simulink model "ElectricVehicleThermalManagementWithHeatPump"  (R2024b)
settings: Solver=VariableStepAuto  StartTime=0.0  StopTime=3600  RelTol=1e-3  AbsTol=1e-3
PreLoadFcn:
  | init_nmpc
InitFcn:
  | init_nmpc
model workspace: external: MATLAB File ElectricVehicleThermalManagementWithHeatPumpParameters.m (data not in the file)
values from neighbouring files (symbols this model uses):
  battery_C1_LUT = [1913.6 12447 30609 ... (first row only)    [ElectricVehicleThermalManagementWithHeatPumpParameters.m]
  battery_capacity_LUT = [280.081 276.25 276.392]    [ElectricVehicleThermalManagementWithHeatPumpParameters.m]
  battery_cell_cp = 795    [ElectricVehicleThermalManagementWithHeatPumpParameters.m]
  battery_cell_mass = 2.5    [ElectricVehicleThermalManagementWithHeatPumpParameters.m]
  battery_Em_LUT = [3.4966 3.5057 3.5148 ... (first row only)    [ElectricVehicleThermalManagementWithHeatPumpParameters.m]
  battery_N_cells = 20    [ElectricVehicleThermalManagementWithHeatPumpParameters.m]
  battery_Qe_init = 0    [ElectricVehicleThermalManagementWithHeatPumpParameters.m]
  battery_R0_LUT = [0.0117 0.0085 0.009 ... (first row only)    [ElectricVehicleThermalManagementWithHeatPumpParameters.m]
  battery_R1_LUT = [0.0109 0.0029 0.0013 ... (first row only)    [ElectricVehicleThermalManagementWithHeatPumpParameters.m]
  battery_SOC_LUT = [0; 0.1; 0.25; 0.5; 0.75; 0.9; 1]    [ElectricVehicleThermalManagementWithHeatPumpParameters.m]
  battery_T_init = -10    [ElectricVehicleThermalManagementWithHeatPumpParameters.m]
  battery_temperature_LUT = [5 20 40]    [ElectricVehicleThermalManagementWithHeatPumpParameters.m]
  cabin_duct_area = 0.04    [ElectricVehicleThermalManagementWithHeatPumpParameters.m]
  cabin_T_init = -10    [ElectricVehicleThermalManagementWithHeatPumpParameters.m]
  chiller_area_primary = 0.43982297150257105    (= 0.439822971503)    [ElectricVehicleThermalManagementWithHeatPumpParameters.m]
  chiller_N_baffles = 3    [ElectricVehicleThermalManagementWithHeatPumpParameters.m]
  chiller_N_tubes = 100    [ElectricVehicleThermalManagementWithHeatPumpParameters.m]
  chiller_tube_D = 0.0035    [ElectricVehicleThermalManagementWithHeatPumpParameters.m]
  chiller_tube_L = 0.4    [ElectricVehicleThermalManagementWithHeatPumpParameters.m]
  chiller_wall_conductivity = 240    [ElectricVehicleThermalManagementWithHeatPumpParameters.m]
  chiller_wall_thickness = 0.0001    [ElectricVehicleThermalManagementWithHeatPumpParameters.m]
  cond_evap_air_area_flow = 0.3906    [ElectricVehicleThermalManagementWithHeatPumpParameters.m]
  cond_evap_air_area_primary = 1.4834999999999998    (= 1.4835)    [ElectricVehicleThermalManagementWithHeatPumpParameters.m]
  cond_evap_W = 0.015    [ElectricVehicleThermalManagementWithHeatPumpParameters.m]
  cond_evap_wall_conductivity = 240    [ElectricVehicleThermalManagementWithHeatPumpParameters.m]
  cond_evap_wall_thickness = 0.0001    [ElectricVehicleThermalManagementWithHeatPumpParameters.m]
  coolant_channel_D = 0.0092    [ElectricVehicleThermalManagementWithHeatPumpParameters.m]
  coolant_pipe_D = 0.019    [ElectricVehicleThermalManagementWithHeatPumpParameters.m]
  coolant_T_init = -10    [ElectricVehicleThermalManagementWithHeatPumpParameters.m]
  coolant_tank_area = 0.0121    [ElectricVehicleThermalManagementWithHeatPumpParameters.m]
  coolant_tank_volume = 1.25    [ElectricVehicleThermalManagementWithHeatPumpParameters.m]
  coolant_valve_D_ratio_max = 0.95    [ElectricVehicleThermalManagementWithHeatPumpParameters.m]
  coolant_valve_D_ratio_min = 0.001    [ElectricVehicleThermalManagementWithHeatPumpParameters.m]
  coolant_valve_displacement = 0.0063    [ElectricVehicleThermalManagementWithHeatPumpParameters.m]
  coolant_valve_S_max = 0.0053    [ElectricVehicleThermalManagementWithHeatPumpParameters.m]
  evaporator_air_area_flow = 0.12    [ElectricVehicleThermalManagementWithHeatPumpParameters.m]
  evaporator_air_area_primary = 0.4323    [ElectricVehicleThermalManagementWithHeatPumpParameters.m]
  evaporator_W = 0.015    [ElectricVehicleThermalManagementWithHeatPumpParameters.m]
  evaporator_wall_conductivity = 240    [ElectricVehicleThermalManagementWithHeatPumpParameters.m]
  evaporator_wall_thickness = 0.0001    [ElectricVehicleThermalManagementWithHeatPumpParameters.m]
  expansion_valve_D_ratio_max = 0.9    [ElectricVehicleThermalManagementWithHeatPumpParameters.m]
  hex_area_primary = 0.070371675440411369    (= 0.0703716754404)    [ElectricVehicleThermalManagementWithHeatPumpParameters.m]
  hex_N_tubes = 64    [ElectricVehicleThermalManagementWithHeatPumpParameters.m]
  hex_tube_D = 0.0035    [ElectricVehicleThermalManagementWithHeatPumpParameters.m]
  hex_wall_conductivity = 240    [ElectricVehicleThermalManagementWithHeatPumpParameters.m]
  hex_wall_thickness = 0.0001    [ElectricVehicleThermalManagementWithHeatPumpParameters.m]
  inner_cond_air_area_flow = 0.1953    [ElectricVehicleThermalManagementWithHeatPumpParameters.m]
  inner_cond_air_area_primary = 0.99520000000000008    (= 0.9952)    [ElectricVehicleThermalManagementWithHeatPumpParameters.m]
  inner_cond_W = 0.02    [ElectricVehicleThermalManagementWithHeatPumpParameters.m]
  inner_cond_wall_conductivity = 240    [ElectricVehicleThermalManagementWithHeatPumpParameters.m]
  inner_cond_wall_thickness = 0.0001    [ElectricVehicleThermalManagementWithHeatPumpParameters.m]
  pump_speed_max = 1000    [ElectricVehicleThermalManagementWithHeatPumpParameters.m]
  radiator_air_area_flow = 0.097499999999999989    (= 0.0975)    [ElectricVehicleThermalManagementWithHeatPumpParameters.m]
  radiator_air_area_primary = 0.43687499999999996    (= 0.436875)    [ElectricVehicleThermalManagementWithHeatPumpParameters.m]
  radiator_W = 0.015    [ElectricVehicleThermalManagementWithHeatPumpParameters.m]
  radiator_wall_conductivity = 240    [ElectricVehicleThermalManagementWithHeatPumpParameters.m]
  radiator_wall_thickness = 0.0001    [ElectricVehicleThermalManagementWithHeatPumpParameters.m]
  refrigerant_p_init = 0.2    [ElectricVehicleThermalManagementWithHeatPumpParameters.m]
  refrigerant_pipe_D = 0.01    [ElectricVehicleThermalManagementWithHeatPumpParameters.m]
  refrigerant_valve_D_ratio_max = 0.95    [ElectricVehicleThermalManagementWithHeatPumpParameters.m]
  refrigerant_valve_displacement = 0.005    [ElectricVehicleThermalManagementWithHeatPumpParameters.m]
libraries: fl_lib x227, nesl_utility x162, SimscapeFluids_lib x30, LiBatteryElements_lib x16, slpidlib x3, SignalEditorBlockLib x1
(part 4 of 13)

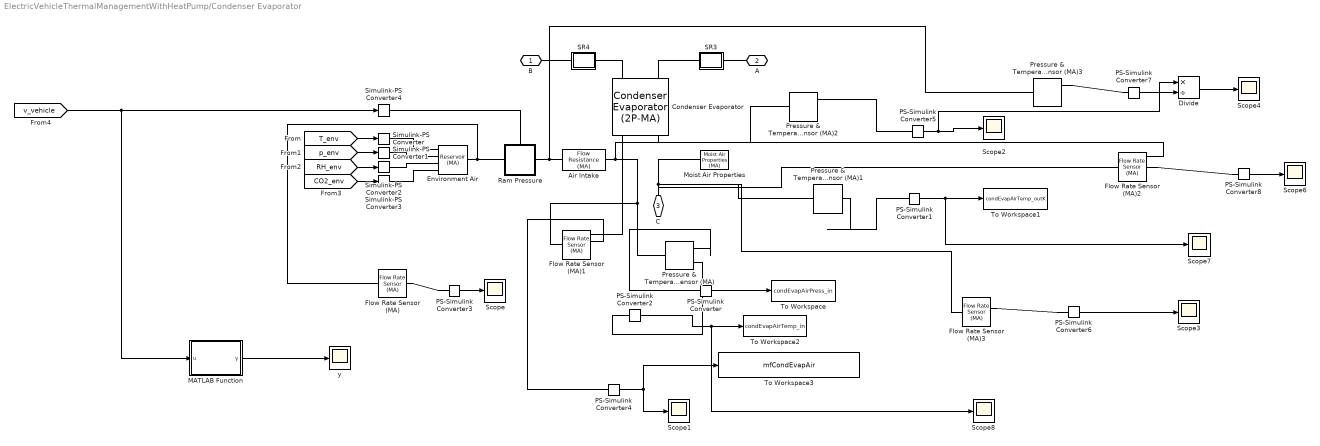
== system ElectricVehicleThermalManagementWithHeatPump/Condenser Evaporator ==
  Air Intake : fl_lib/Moist Air/Elements/Flow Resistance (MA)  delta_p_nominal=5e-4 MPa  mdot_nominal=1 kg/s  rho_nominal=1.2 kg/m^3  area=cabin_duct_area m^2  laminar_fraction=1e-3
  Condenser Evaporator : SimscapeFluids_lib/Heat Exchangers/Two-Phase Fluid - Moist Air/Condenser Evaporator (2P-MA)  flow_arrangement=fluids.heat_exchangers.enum.FlowArrangement2PMA.Cross  cross_flow_arrangement=fluids.heat_exchangers.enum.CrossFlowArrangement2PMA.UnmixedUnmixed  R_wall=cond_evap_wall_thickness / cond_evap_air_area_primary / cond_evap_wall_conductivity K/W  area_A1=pi * refrigerant_pipe_D^2 / 4 m^2  area_B1=pi * refrigerant_pipe_D^2 / 4 m^2  area_A2=cabin_duct_area m^2  area_B2=cabin_duct_area m^2  tube_num_2P=cond_evap_N_tubes  tube_length_2P=cond_evap_L m  tube_cross_section_2P=fluids.heat_exchangers.enum.TubeCrossSection.Rectangular  tube_diameter_2P=0.1 m  tube_width_2P=cond_evap_W m  tube_height_2P=cond_evap_tube_H m  tube_inner_diameter_2P=0.05 m  tube_outer_diameter_2P=0.1 m  tube_flow_area_2P=0.01 m^2  tube_wetted_perimeter_2P=0.4 m  tube_heat_perimeter_2P=0.4 m  tube_pressure_loss_spec_2P=fluids.heat_exchangers.enum.TubePressureLossSpec2P.Haaland  tube_loss_coeff_2P=10  tube_local_pressure_loss_spec_2P=fluids.heat_exchangers.enum.LocalLossSpec.AggregateLength  tube_length_add_2P=cond_evap_tube_Leq m  tube_local_loss_coefficient_2P=0.1  tube_roughness_pressure_2P=15e-6 m  tube_Re_lam_pressure_2P=2000  tube_Re_tur_pressure_2P=4000  tube_shape_factor_generic_2P=64  tube_heat_coeff_spec_2P=fluids.heat_exchangers.enum.TubeHeatCoeffSpec2P.GneilinskiCavalliniZecchin  tube_colburn_coeff_liq_2P=[.023, .8, .33]  tube_colburn_coeff_mix_2P=[.05, .8, .33]  tube_colburn_coeff_vap_2P=[.023, .8, .33]  tube_roughness_heat_2P=15e-6 m  tube_Re_lam_heat_2P=2000  tube_Re_tur_heat_2P=4000  tube_Nu_lam_generic_2P=3.66  fouling_factor_2P=0.1 m^2*K/kW  fin_area_2P=cond_evap_tube_area_webs m^2  fin_efficiency_2P=0.6  energy_spec_2P=foundation.enum.energy_spec.void_fraction  p_init_2P=refrigerant_p_init MPa  T_init_2P=293.15 K  x_init_2P=0.5  alpha_init_2P=refrigerant_alpha_init  h_init_2P=1500 kJ/kg  u_init_2P=1500 kJ/kg  flow_geometry_MA=fluids.heat_exchangers.enum.FlowGeometryMA.Generic  tube_num_MA=1  tube_length_MA=5 m  tube_cross_section_MA=fluids.heat_exchangers.enum.TubeCrossSection.Circular  tube_diameter_MA=0.1 m  tube_width_MA=0.1 m  tube_height_MA=0.1 m  tube_inner_diameter_MA=0.05 m  tube_outer_diameter_MA=0.1 m  tube_flow_area_MA=0.01 m^2  tube_wetted_perimeter_MA=0.4 m  tube_heat_perimeter_MA=0.4 m  tube_pressure_loss_spec_MA=fluids.heat_exchangers.enum.TubePressureLossSpec.Haaland  tube_loss_coeff_MA=10  tube_local_pressure_loss_spec_MA=fluids.heat_exchangers.enum.LocalLossSpec.AggregateLength  tube_length_add_MA=0.1 m  tube_local_loss_coefficient_MA=0.1  tube_roughness_pressure_MA=15e-6 m  tube_Re_lam_pressure_MA=2000  tube_Re_tur_pressure_MA=4000  tube_shape_factor_generic_MA=64  tube_heat_coeff_spec_MA=fluids.heat_exchangers.enum.TubeHeatCoeffSpec.Gneilinski  tube_colburn_coeff_MA=[.023, .8, .33]  tube_roughness_heat_MA=15e-6 m  tube_Re_lam_heat_MA=2000  tube_Re_tur_heat_MA=4000  tube_Nu_lam_generic_MA=3.66  bank_arrangement_MA=fluids.heat_exchangers.enum.BankArrangement.Inline  bank_num_rows_MA=5  bank_tubes_per_row_MA=5  bank_width_MA=1 m  bank_tube_diameter_MA=0.05 m  bank_longitudinal_pitch_MA=0.15 m  bank_transverse_pitch_MA=0.15 m  bank_pressure_loss_spec_MA=fluids.heat_exchangers.enum.BankPressureLossSpec.Martin  bank_euler_MA=10  bank_heat_coeff_spec_MA=fluids.heat_exchangers.enum.BankHeatCoeffSpec.Martin  bank_colburn_coeff_MA=[.27, .63, .36]  generic_flow_area_MA=cond_evap_air_area_flow m^2  generic_heat_area_MA=cond_evap_air_area_primary m^2  generic_volume_MA=cond_evap_air_area_flow * cond_evap_W m^3  generic_loss_coeff_MA=10  generic_colburn_coeff_MA=[0.27, 0.63, 0.36]  fouling_factor_MA=0.1 m^2*K/kW  fin_area_MA=cond_evap_air_area_fins m^2  fin_efficiency_MA=0.7  p_init_MA=cabin_p_init MPa  T_init_MA=cabin_T_init degC  humidity_spec_MA=foundation.enum.HumiditySpec.RelativeHumidity  RH_init_MA=cabin_RH_init  x_w_init_MA=0.01  y_w_init_MA=0.01  HR_init_MA=0.01  Tw_init_MA=287 K  trace_gas_spec_MA=foundation.enum.trace_gas_spec.mole_fraction  x_g_init_MA=0.001  y_g_init_MA=cabin_CO2_init  r_d_init_MA=0  RH_ws_MA=1  time_constant_cond_MA=1e-3 s  time_constant_evap_MA=1e-3 s  fraction_entrained_MA=1
      settings: InternalSimscapePortConfiguration="{\"Bottom\":[],\"Left\":[{\"id\":\"A1\",\"label\":\"A1\",\"type\":\"foundation.two_phase_fluid.two_phase_fluid\"},{\"id\":\"Z\",\"label\":\"Z\",\"type\":\"output\"},{\"id\":\"B1\",\"label\":\"B1\",\"type\":\"foundation.two_phase_fluid.two_phase_fluid\"}],\"Right\":[{\"id\":\"A2\",\"label\":\"A2\",\"type\":\"foundation.moist_air.moist_air\"},{\"id\":\"W\",\"label\":\"W\",\"type\":\"output\"},{\"id\":\"B2\",\"label\":\"B2\",\"type\":\"foundation.moist_air.moist_air\"}],\"Top\":[]}"
  Divide : Product  Inputs=*/
  Environment Air : fl_lib/Moist Air/Elements/Reservoir (MA)  pressure_input=true  pressure_spec=foundation.enum.pressure_spec.atmospheric  reservoir_pressure=0.101325 MPa  temperature_input=true  temperature_spec=foundation.enum.temperature_spec.atmospheric  reservoir_temperature=293.15 K  humidity_input=true  humidity_spec=foundation.enum.HumiditySpec.RelativeHumidity  reservoir_RH=0.5  reservoir_x_w=0.01  reservoir_y_w=0.01  reservoir_HR=0.01  reservoir_Tw=287 K  trace_gas_input=true  trace_gas_spec=foundation.enum.trace_gas_spec.mole_fraction  reservoir_x_g=0.001  reservoir_y_g=0.001  water_droplets_input=false  reservoir_r_d=0  RH_ws=1  area_A=cabin_duct_area m^2  input_error_spec=foundation.enum.input_range_error.warn
      settings: InternalSimscapePortConfiguration="{\"Bottom\":[],\"Left\":[{\"id\":\"A\",\"label\":\"A\",\"type\":\"foundation.moist_air.moist_air\"}],\"Right\":[{\"id\":\"T\",\"label\":\"T\",\"type\":\"input\"},{\"id\":\"P\",\"label\":\"P\",\"type\":\"input\"},{\"id\":\"W\",\"label\":\"W\",\"type\":\"input\"},{\"id\":\"G\",\"label\":\"G\",\"type\":\"input\"}],\"Top\":[]}"
  Flow Rate Sensor (MA) : fl_lib/Moist Air/Sensors/Flow Rate Sensor (MA)  mass_flow_measure=true  volumetric_flow_measure=false  volumetric_flow_conditions=foundation.enum.volumetric_flow_conditions.actual  p_std=0.101325 MPa  T_std=20 degC  RH_std=0.65  energy_flow_measure=true  vapor_flow_measure=false  gas_flow_measure=false  droplets_flow_measure=false
      settings: InternalSimscapePortConfiguration="{\"Bottom\":[{\"id\":\"PHI\",\"label\":\"φ\",\"type\":\"output\"}],\"Left\":[{\"id\":\"A\",\"label\":\"A\",\"type\":\"foundation.moist_air.moist_air\"}],\"Right\":[{\"id\":\"B\",\"label\":\"B\",\"type\":\"foundation.moist_air.moist_air\"},{\"id\":\"M\",\"label\":\"M\",\"type\":\"output\"}],\"Top\":[]}"
  Flow Rate Sensor (MA)1 : fl_lib/Moist Air/Sensors/Flow Rate Sensor (MA)  mass_flow_measure=true  volumetric_flow_measure=true  volumetric_flow_conditions=foundation.enum.volumetric_flow_conditions.actual  p_std=0.101325 MPa  T_std=20 degC  RH_std=0.65  energy_flow_measure=true  vapor_flow_measure=false  gas_flow_measure=false  droplets_flow_measure=false
      settings: InternalSimscapePortConfiguration="{\"Bottom\":[{\"id\":\"PHI\",\"label\":\"φ\",\"type\":\"output\"}],\"Left\":[{\"id\":\"A\",\"label\":\"A\",\"type\":\"foundation.moist_air.moist_air\"}],\"Right\":[{\"id\":\"B\",\"label\":\"B\",\"type\":\"foundation.moist_air.moist_air\"},{\"id\":\"M\",\"label\":\"M\",\"type\":\"output\"},{\"id\":\"V\",\"label\":\"V\",\"type\":\"output\"}],\"Top\":[]}"
  Flow Rate Sensor (MA)2 : fl_lib/Moist Air/Sensors/Flow Rate Sensor (MA)  mass_flow_measure=true  volumetric_flow_measure=false  volumetric_flow_conditions=foundation.enum.volumetric_flow_conditions.actual  p_std=0.101325 MPa  T_std=20 degC  RH_std=0.65  energy_flow_measure=true  vapor_flow_measure=false  gas_flow_measure=false  droplets_flow_measure=false
      settings: InternalSimscapePortConfiguration="{\"Bottom\":[{\"id\":\"PHI\",\"label\":\"φ\",\"type\":\"output\"}],\"Left\":[{\"id\":\"A\",\"label\":\"A\",\"type\":\"foundation.moist_air.moist_air\"}],\"Right\":[{\"id\":\"B\",\"label\":\"B\",\"type\":\"foundation.moist_air.moist_air\"},{\"id\":\"M\",\"label\":\"M\",\"type\":\"output\"}],\"Top\":[]}"
  Flow Rate Sensor (MA)3 : fl_lib/Moist Air/Sensors/Flow Rate Sensor (MA)  mass_flow_measure=true  volumetric_flow_measure=true  volumetric_flow_conditions=foundation.enum.volumetric_flow_conditions.actual  p_std=0.101325 MPa  T_std=20 degC  RH_std=0.65  energy_flow_measure=true  vapor_flow_measure=false  gas_flow_measure=false  droplets_flow_measure=false
      settings: InternalSimscapePortConfiguration="{\"Bottom\":[{\"id\":\"PHI\",\"label\":\"φ\",\"type\":\"output\"}],\"Left\":[{\"id\":\"A\",\"label\":\"A\",\"type\":\"foundation.moist_air.moist_air\"}],\"Right\":[{\"id\":\"B\",\"label\":\"B\",\"type\":\"foundation.moist_air.moist_air\"},{\"id\":\"M\",\"label\":\"M\",\"type\":\"output\"},{\"id\":\"V\",\"label\":\"V\",\"type\":\"output\"}],\"Top\":[]}"
  MATLAB Function : MATLAB Function  TreatAsAtomicUnit=on
  Moist Air Properties : fl_lib/Moist Air/Utilities/Moist Air Properties (MA)  R_a=287.047 J/(K*kg)  T_TLU=[-56.55, -50 : 10 : -10, -5 : 1 : 5, 10 : 10 : 350]' degC  h_a_TLU=[342.414066793634; 349.003411914139; 359.061417476782; 369.117728274935; 379.173188407993; 389.228602960013; 394.256538873206; 395.262156814682; 396.26778682262; 397.27342967397; 398.279086145689; 399.284757014822; 400.290443058569; 401.296145054364; 402.301863779931; 403.307600013352; 404.313354533128; 409.342428711098; 419.402397945314; 429.465451846544; 439.532387826623; 449.604014793745; 459.68115297076; 469.764632657687; 479.855292205971; 489.953975419749; 500.06152856014; 510.178797098051; 520.306622336267; 530.445838000969; 540.597266885076; 550.761717610289; 560.939981561004; 571.132830031086; 581.341011613777; 591.565249855533; 601.806241186423; 612.064653132654; 622.341122810862; 632.636255698901; 642.95062467384; 653.284769304793; 663.639195385783; 674.014374692179; 684.410744943084; 694.828709951456; 705.268639943519; 715.730872029167; 726.215710805484; 736.723429076127; 747.254268670154; 757.808441344776] kJ/kg  mu_a_TLU=[14.2568884161326; 14.6140128551699; 15.151727785151; 15.6806860927178; 16.201235181264; 16.7137043838401; 16.9670072430524; 17.017438132541; 17.0677931537044; 17.1180726001803; 17.1682767640582; 17.2184059358881; 17.2684604046898; 17.318440457962; 17.3683463816913; 17.4181784603614; 17.467936976962; 17.7156359301048; 18.2056752419787; 18.6887904184394; 19.1652345249932; 19.6352479488881; 20.099059157425; 20.5568854116507; 21.008933436444; 21.4554000485251; 21.8964727442509; 22.3323302492491; 22.7631430320408; 23.1890737838183; 23.6102778665211; 24.0269037312887; 24.4390933092858; 24.8469823767971; 25.2507008963847; 25.6503733357905; 26.0461189661617; 26.438052141067; 26.8262825576728; 27.210915501349; 27.5920520748824; 27.969789413389; 28.3442208859359; 28.7154362848061; 29.0835220032714; 29.4485612026716; 29.8106339695395; 30.169817463453; 30.5261860562487; 30.8798114631771; 31.2307628665438; 31.5791070323335] s*uPa  k_a_TLU=[19.8808491891482; 20.4162457047568; 21.2248745869044; 22.0232455041378; 22.8117316528767; 23.59069155438; 23.9767077285082; 24.0536401764626; 24.130482853517; 24.2072360894785; 24.2839002127411; 24.3604755502875; 24.4369624276914; 24.5133611691197; 24.5896720973349; 24.6658955336975; 24.7420317981691; 25.1214166432482; 25.8738284673185; 26.6180151791963; 27.3542675863918; 28.0828636150405; 28.8040688184917; 29.5181369069754; 30.2253102842368; 30.9258205811167; 31.6198891790667; 32.307727718801; 32.989538590917; 33.6655154065126; 34.3358434467079; 35.0007000906151; 35.6602552217624; 36.314671613305; 36.9641052925838; 37.6087058857479; 38.2486169432557; 38.8839762471259; 39.5149161008418; 40.1415636028127; 40.7640409042923; 41.3824654526272; 41.9969502206863; 42.6076039232795; 43.2145312213471; 43.8178329146528; 44.4176061236819; 45.0139444614019; 45.6069381955058; 46.1966744017242; 46.7832371087507; 47.3667074352967] mW/(K*m)  p_min=1 kPa  p_max=inf MPa  T_min=-56.55 degC  T_max=350 degC  properties_range_check=simscape.enum.assert.action.error  p_atm=0.101325 MPa  T_atm=20 degC  enable_droplets=false  R_w=461.523 J/(K*kg)  p_ws_TLU=[1.71168953425982e-06; 3.93770601979424e-06; 1.28411717710344e-05; 3.80051394873809e-05; .00010323902900209; .000259873810798063; .000401741022116384; .000437454836117844; .000476040820618202; .000517704666185737; .000562664883741207; .000611212677444345; .000657085634113763; .000705985593917791; .00075808051438111; .000813548355379396; .000872575113841924; .00122819910164487; .00233931836947519; .00424697076171126; .00738493802968097; .012351945812707; .0199464343236764; .0312009300307261; .0474144740241604; .0701817658485933; .101417996663294; .143378712947169; .198674420476403; .270279976781692; .361539099388177; .476164537971214; .618234621423587; .792187006980199; 1.00281053608169; 1.25523615516845; 1.55492790046272; 1.90767499353199; 2.31958617020155; 2.79708749692822; 3.34692514426746; 3.97617493064794; 4.69226099229504; 5.50298678300951; 6.41658290952841; 7.44177834442093; 8.58790494083256; 9.86505121117553; 11.284292927457; 12.8580516000122; 14.6006773719404; 16.5294151389953] MPa  h_w_vap_TLU=[2836.88241275372; 2837.81392500514; 2838.63937175807; 2838.7309929628; 2838.06905313927; 2836.62597341095; 2835.60023952573; 2835.37006381376; 2835.13143158077; 2834.88429145066; 2834.62859062897; 2500.93420564316; 2498.55452890293; 2496.17317793437; 2493.7941260618; 2491.41713708944; 2489.04199020767; 2477.18706302224; 2453.51925941961; 2429.81122987564; 2405.97728678685; 2381.94712654051; 2357.65452030374; 2333.03120800924; 2308.00352809267; 2282.49062771796; 2256.40372152657; 2229.64615315163; 2202.11407337172; 2173.6974807639; 2144.28128268553; 2113.74600964951; 2081.9678834089; 2048.81807129851; 2014.16109962579; 1977.85249331179; 1939.73572816654; 1899.63852389863; 1857.36838273035; 1812.70710332357; 1765.4037880462; 1715.16561416478; 1661.64526339623; 1604.4232249434; 1542.98206457018; 1476.66790089115; 1404.63083498414; 1325.72875296442; 1238.36212284382; 1140.16281350074; 1027.31658328826; 892.746804215825] kJ/kg  h_w_TLU=[2396.53078650168; 2408.65722023252; 2427.16766028467; 2445.66624034104; 2464.1379798878; 2482.5594701893; 2491.7412703989; 2493.57467660537; 2495.40699233755; 2497.23816944599; 2499.06815833272; 2500.89261781717; 2502.73123919979; 2504.56496564907; 2506.39800457704; 2508.23033644628; 2510.06194120626; 2519.20831890725; 2537.43340437276; 2555.54520329515; 2573.51032237465; 2591.28888786817; 2608.83487221908; 2626.09640083333; 2643.01588134754; 2659.53001419864; 2675.5827869577; 2696.18462565746; 2716.49989554204; 2736.6235211014; 2756.61216047677; 2776.50561774616; 2796.33378923373; 2816.11979584021; 2835.88181424959; 2855.6343057571; 2875.38889328914; 2895.15500578618; 2914.94035966265; 2934.75132291939; 2954.59319332093; 2974.47041287496; 2994.38673461102; 3014.34535330297; 3034.34900869544; 3054.40006758361; 3074.50058949656; 3094.65237956705; 3114.85703131193; 3135.11596141057; 3155.43043809331; 3175.80160439414] kJ/kg  mu_w_TLU=[6.9886414857741; 7.21462000349698; 7.55962537406626; 7.90463074463554; 8.24963611520482; 8.5946414857741; 8.76714417105874; 8.80164470811567; 8.8361452451726; 8.87064578222952; 8.90514631928645; 8.93964685634338; 8.97414739340031; 9.00294911497154; 9.0318980288863; 9.06099135942002; 9.09022638806001; 9.23843559844524; 9.5440595677542; 9.86015858692705; 10.1848429274122; 10.5164578096049; 10.8535319382781; 11.1947482575333; 11.5389294976352; 11.8850331780701; 12.2322493177351; 12.6188533568459; 13.0082793358938; 13.4003380262893; 13.7948421428098; 14.1916095618232; 14.590464747099; 14.9912394314964; 15.3937729006119; 15.7979120385447; 16.203511226482; 16.610432150303; 17.0185435533718; 17.4277209582061; 17.8378463726577; 18.2488079909412; 18.6604998963166; 19.0728217698535; 19.485678608085; 19.8989804512625; 20.3126421231677; 20.7265829829225; 21.1407266888906; 21.5550009745266; 21.969337435876; 22.3836713303269] s*uPa  k_w_TLU=[12.4916816538045; 12.9847788176262; 13.737598915064; 14.4904190125018; 15.2432391099396; 15.9960592073774; 16.3724692560963; 16.4477512658401; 16.5230332755839; 16.5983152853277; 16.6735972950715; 16.7488793048152; 16.824161314559; 16.8886088206517; 16.9532779906513; 17.0181691764255; 17.083282769915; 17.4122036181723; 18.0870861656185; 18.7855813517187; 19.5093466408385; 20.2607864040347; 21.0430876297671; 21.8602068151121; 22.7168164077153; 23.6182141540994; 24.5698636875305; 25.4024944426483; 26.2458938647479; 27.1009155051916; 27.968142896353; 28.8479507975112; 29.7405485790829; 30.646029672269; 31.5643932662527; 32.4955693285114; 33.4394360046859; 34.3958329885356; 35.3645718140131; 36.3454437886179; 37.3382261129791; 38.3426866012072; 39.3585873185985; 40.3856873794121; 41.4237450915028; 42.4725195920623; 43.5317720862424; 44.6012667755489; 45.6807715437344; 46.7700584531355; 47.8689040929333; 48.9770898119082] mW/(K*m)  D_w=25 mm^2/s  trace_gas_model=foundation.enum.trace_gas_model.track_fraction  R_g=188.923 J/(K*kg)  h_g_TLU=[439.555216276024; 444.670268214299; 452.538618857965; 460.487124266174; 468.522588773143; 476.64941595933; 480.747985385885; 481.570543185868; 482.394052396612; 483.218514286302; 484.043930026094; 484.87030069324; 485.697627274149; 486.525910667382; 487.355151686572; 488.185351063277; 489.016509449741; 493.186704132078; 501.599194941473; 510.107689945701; 518.711611059603; 527.410026767716; 536.20176474847; 545.085474167968; 554.059675464379; 563.122805439004; 572.273250917104; 581.509372969931; 590.829525041787; 600.232066635428; 609.715373504524; 619.277845094572; 628.91790983254; 638.634028741375; 648.424697754692; 658.288449028076; 668.22385148184; 678.229510761734; 688.30406876583; 698.446202855373; 708.654624842952; 718.928079831753; 729.265344963773; 739.665228122078; 750.126566621791; 760.648225916092; 771.229098336723; 781.86810188302; 792.564179069104; 803.316295835373; 814.123440527678; 824.984622945405] kJ/kg  mu_g_TLU=[10.9386626034033; 11.2618160869372; 11.7542862475187; 12.2454955799777; 12.7352208796158; 13.2232325321233; 13.4665248390743; 13.5151226761166; 13.5636997995993; 13.6122559954699; 13.6607910510226; 13.709304754931; 13.757796897279; 13.8062672695897; 13.8547156648526; 13.9031418775498; 13.9515457036801; 14.1932220047332; 14.6747828595747; 15.153802214283; 15.6301123398299; 16.1035631756244; 16.574022106427; 17.0413733976215; 17.5055174102327; 17.9663696812767; 18.4238599299346; 18.8779310322956; 19.3285379947687; 19.7756469471288; 20.2192341695255; 20.6592851629269; 21.0957937689132; 21.5287613421341; 21.9581959768344; 22.3841117874779; 22.8065282425078; 23.2254695495877; 23.6409640901974; 24.0530439011453; 24.4617442003854; 24.8671029544344; 25.269160484669; 25.6679591098169; 26.0635428220247; 26.4559569939835; 26.8452481147025; 27.2314635516519; 27.6146513371198; 27.9948599767665; 28.3721382784874; 28.74653519983] s*uPa  k_g_TLU=[10.7373095949238; 11.1772934980884; 11.862915506018; 12.5638333280734; 13.2785475592421; 14.005722199619; 14.3736017704762; 14.4475028211958; 14.5215096973787; 14.5956213250986; 14.6698366403414; 14.7441545888563; 14.8185741260114; 14.8930942166532; 14.9677138349692; 15.0424319643548; 15.1172475972825; 15.4927536712633; 16.2505237772467; 17.0165521650722; 17.7899991951805; 18.5700903932503; 19.3561099002839; 20.1473949639617; 20.9433312278214; 21.7433486448307; 22.5469178892132; 23.3535471729555; 24.1627793965491; 24.9741895799701; 25.7873825314493; 26.6019907190427; 27.4176723115859; 28.2341093347412; 29.0510055857402; 29.8680879651392; 30.6851034165693; 31.5018116707882; 32.3179924018673; 33.1334410491403; 33.9479677779769; 34.7613965127281; 35.5735640361829; 36.3843191504339; 37.1935218945334; 38.0010428147395; 38.80676228352; 39.6105698638057; 40.412363715274; 41.2120500397018; 42.0095425626597; 42.8047620490288] mW/(K*m)  D_g=16 mm^2/s
  PS-Simulink Converter{,1..8} (9 alike) : nesl_utility/PS-Simulink Converter  PhysicalDomain=network_engine_domain  SubClassName=ps_output  LeftPortType=input  RightPortType=output  PseudoPeriodic=off  Frequencies=[]  VectorFormat=inherit  Unit=inherit  AffineConversion=off
  Pressure & Temperature Sensor (MA) : fl_lib/Moist Air/Sensors/Pressure & Temperature Sensor (MA)  reference=foundation.enum.MeasurementReference.absolute  pressure=true  pressure_spec=foundation.enum.PressureMeasementSpec.Absolute  temperature=true
      settings: InternalSimscapePortConfiguration="{\"Bottom\":[{\"id\":\"T\",\"label\":\"T\",\"type\":\"output\"}],\"Left\":[{\"id\":\"A\",\"label\":\"A\",\"type\":\"foundation.moist_air.moist_air\"}],\"Right\":[{\"id\":\"Pa\",\"label\":\"Pa\",\"type\":\"output\"}],\"Top\":[]}"
  Pressure & Temperature Sensor (MA)1 : fl_lib/Moist Air/Sensors/Pressure & Temperature Sensor (MA)  reference=foundation.enum.MeasurementReference.absolute  pressure=false  pressure_spec=foundation.enum.PressureMeasementSpec.Absolute  temperature=true
      settings: InternalSimscapePortConfiguration="{\"Bottom\":[{\"id\":\"T\",\"label\":\"T\",\"type\":\"output\"}],\"Left\":[{\"id\":\"A\",\"label\":\"A\",\"type\":\"foundation.moist_air.moist_air\"}],\"Right\":[],\"Top\":[]}"
  Pressure & Temperature Sensor (MA)2 : fl_lib/Moist Air/Sensors/Pressure & Temperature Sensor (MA)  reference=foundation.enum.MeasurementReference.absolute  pressure=true  pressure_spec=foundation.enum.PressureMeasementSpec.Absolute  temperature=true
      settings: InternalSimscapePortConfiguration="{\"Bottom\":[{\"id\":\"T\",\"label\":\"T\",\"type\":\"output\"}],\"Left\":[{\"id\":\"A\",\"label\":\"A\",\"type\":\"foundation.moist_air.moist_air\"}],\"Right\":[{\"id\":\"Pa\",\"label\":\"Pa\",\"type\":\"output\"}],\"Top\":[]}"
  Pressure & Temperature Sensor (MA)3 : fl_lib/Moist Air/Sensors/Pressure & Temperature Sensor (MA)  reference=foundation.enum.MeasurementReference.absolute  pressure=true  pressure_spec=foundation.enum.PressureMeasementSpec.Absolute  temperature=true
      settings: InternalSimscapePortConfiguration="{\"Bottom\":[{\"id\":\"T\",\"label\":\"T\",\"type\":\"output\"}],\"Left\":[{\"id\":\"A\",\"label\":\"A\",\"type\":\"foundation.moist_air.moist_air\"}],\"Right\":[{\"id\":\"Pa\",\"label\":\"Pa\",\"type\":\"output\"}],\"Top\":[]}"
  Ram Pressure : Subsystem
      settings: PortSchema="{\"entries\":[{\"content\":{\"sides\":[{\"content\":{\"connectorIds\":[\"LConn1\"]},\"type\":\"ConnectorPlacement.EquallySpacedRectSide\",\"uuid\":\"75e3029b-49fb-4aa2-a270-5647ec8f7cc2\"},{\"content\":{\"connectorIds\":[\"RConn1\"],\"side\":\"RIGHT\"},\"type\":\"ConnectorPlacement.EquallySpacedRectSide\",\"uuid\":\"a5773782-5ea1-4526-866f-91c4aa99dd69\"},{\"content\":{\"connectorIds\":[\"LConn2\"],\"side\":\"TOP\"},\"type\":\"ConnectorPlacement.EquallySpacedRectSide\",\"uuid\":\"b1426a6c-920c-4fe3-a6f1-49137f31d8b5\"}]},\"type\":\"ConnectorPlacement.EquallySpacedConnector\",\"uuid\":\"8a57436c-822b-4551-8b15-f9c616e1048b\"}],\"packageUris\":[\"http://schema.mathworks.com/mf0/Connector/R2020b\"],\"version\":\"1.0\"}"
  SR3 : Subsystem
  SR4 : Subsystem
  Scope{,1..4,6..8} (8 alike) : Scope
  Simulink-PS Converter : nesl_utility/Simulink-PS Converter  PhysicalDomain=network_engine_domain  SubClassName=ps_input  LeftPortType=input  RightPortType=output  PseudoPeriodic=off  Frequencies=[]  NoiseDistribution=none  NoiseParameters=[]  Unit=degC  AffineConversion=on  FilteringAndDerivatives=provide  SimscapeFilterOrder=1  InputFilterTimeConstant=0.001  UdotUserProvided=0
  Simulink-PS Converter1 : nesl_utility/Simulink-PS Converter  PhysicalDomain=network_engine_domain  SubClassName=ps_input  LeftPortType=input  RightPortType=output  PseudoPeriodic=off  Frequencies=[]  NoiseDistribution=none  NoiseParameters=[]  Unit=MPa  AffineConversion=off  FilteringAndDerivatives=provide  SimscapeFilterOrder=1  InputFilterTimeConstant=0.001  UdotUserProvided=0
  Simulink-PS Converter2 : nesl_utility/Simulink-PS Converter  PhysicalDomain=network_engine_domain  SubClassName=ps_input  LeftPortType=input  RightPortType=output  PseudoPeriodic=off  Frequencies=[]  NoiseDistribution=none  NoiseParameters=[]  Unit=1  AffineConversion=off  FilteringAndDerivatives=provide  SimscapeFilterOrder=1  InputFilterTimeConstant=0.001  UdotUserProvided=0
  Simulink-PS Converter3 : nesl_utility/Simulink-PS Converter  PhysicalDomain=network_engine_domain  SubClassName=ps_input  LeftPortType=input  RightPortType=output  PseudoPeriodic=off  Frequencies=[]  NoiseDistribution=none  NoiseParameters=[]  Unit=1  AffineConversion=off  FilteringAndDerivatives=provide  SimscapeFilterOrder=1  InputFilterTimeConstant=0.001  UdotUserProvided=0
  Simulink-PS Converter4 : nesl_utility/Simulink-PS Converter  PhysicalDomain=network_engine_domain  SubClassName=ps_input  LeftPortType=input  RightPortType=output  PseudoPeriodic=off  Frequencies=[]  NoiseDistribution=none  NoiseParameters=[]  Unit=km/hr  AffineConversion=off  FilteringAndDerivatives=provide  SimscapeFilterOrder=1  InputFilterTimeConstant=0.001  UdotUserProvided=0
  To Workspace : ToWorkspace  VariableName=condEvapAirPress_in  SampleTime=-1
  To Workspace1 : ToWorkspace  VariableName=condEvapAirTemp_outK  SampleTime=-1
  To Workspace2 : ToWorkspace  VariableName=condEvapAirTemp_in  SampleTime=-1
  To Workspace3 : ToWorkspace  VariableName=mfCondEvapAir  SampleTime=-1
  y : Scope
  B : PMIOPort  Side=Left
  A : PMIOPort  Port=2  Side=Right
  C : PMIOPort  Port=3  Side=Right
  wires:
  [RH_env] -> Simulink-PS Converter2/1
  [CO2_env] -> Simulink-PS Converter3/1
  [T_env] -> Simulink-PS Converter/1
  [p_env] -> Simulink-PS Converter1/1
  [v_vehicle] -> MATLAB Function/1(u), Simulink-PS Converter4/1
  PS-Simulink Converter/1 -> To Workspace/1
  PS-Simulink Converter1/1 -> Scope7/1, To Workspace1/1
  PS-Simulink Converter2/1 -> Scope8/1, To Workspace2/1
  PS-Simulink Converter3/1 -> Scope/1
  PS-Simulink Converter4/1 -> Scope1/1, To Workspace3/1
  PS-Simulink Converter6/1 -> Scope3/1
  PS-Simulink Converter5/1 -> Divide/1, Scope2/1
  PS-Simulink Converter7/1 -> Divide/2
  Divide/1 -> Scope4/1
  MATLAB Function/1(y) -> y/1
  PS-Simulink Converter8/1 -> Scope6/1
  connections:
  Pressure & Temperature Sensor (MA)1/LConn1 -- Flow Rate Sensor (MA)3/LConn1 -- Moist Air Properties/RConn1 -- Flow Rate Sensor (MA)2/LConn1 -- C/RConn1
  Air Intake/RConn1 -- Pressure & Temperature Sensor (MA)2/LConn1 -- Pressure & Temperature Sensor (MA)/LConn1 -- Flow Rate Sensor (MA)1/LConn1
  SR3/LConn1 -- A/RConn1
  Simulink-PS Converter/RConn1 -- Environment Air/RConn1
  Simulink-PS Converter2/RConn1 -- Environment Air/RConn3
  Ram Pressure/RConn1 -- Pressure & Temperature Sensor (MA)3/LConn1 -- Air Intake/LConn1
  Simulink-PS Converter1/RConn1 -- Environment Air/RConn2
  SR4/LConn1 -- Condenser Evaporator/LConn3
  SR3/RConn1 -- Condenser Evaporator/LConn1
  Ram Pressure/LConn1 -- Flow Rate Sensor (MA)/LConn1 -- Environment Air/LConn1
  Simulink-PS Converter4/RConn1 -- Ram Pressure/LConn2
  Simulink-PS Converter3/RConn1 -- Environment Air/RConn4
  SR4/RConn1 -- B/RConn1
  PS-Simulink Converter/LConn1 -- Pressure & Temperature Sensor (MA)/RConn1
  PS-Simulink Converter1/LConn1 -- Pressure & Temperature Sensor (MA)1/RConn1
  PS-Simulink Converter2/LConn1 -- Pressure & Temperature Sensor (MA)/RConn2
  PS-Simulink Converter3/LConn1 -- Flow Rate Sensor (MA)/RConn2
  PS-Simulink Converter6/LConn1 -- Flow Rate Sensor (MA)3/RConn2
  Flow Rate Sensor (MA)1/RConn2 -- PS-Simulink Converter4/LConn1
  Flow Rate Sensor (MA)1/RConn1 -- Condenser Evaporator/RConn3
  PS-Simulink Converter5/LConn1 -- Pressure & Temperature Sensor (MA)2/RConn1
  Pressure & Temperature Sensor (MA)3/RConn1 -- PS-Simulink Converter7/LConn1
  Flow Rate Sensor (MA)2/RConn1 -- Condenser Evaporator/RConn1
  Flow Rate Sensor (MA)2/RConn2 -- PS-Simulink Converter8/LConn1

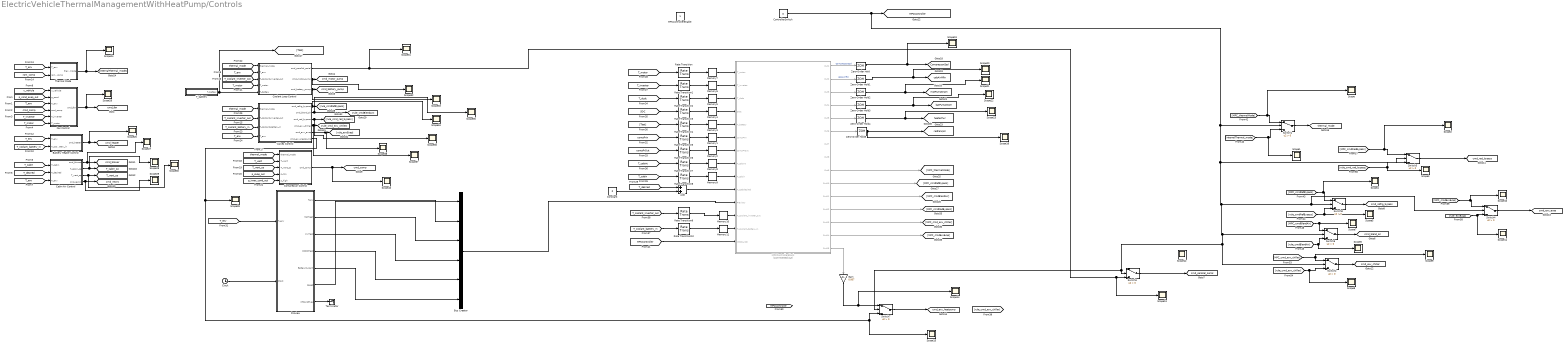
== system ElectricVehicleThermalManagementWithHeatPump/Controls ==
  Add : Sum
  Battery Heater Control : Subsystem
  Bus Creator : BusCreator  Inputs=6
  Cabin Air Control : Subsystem
  Clock : Clock
  Compressor Control : Subsystem
  Constant : Constant  Value=0
  ControllerSwitch : Constant  Value=0
  Coolant Loop Control : Subsystem
  Fan Control : Subsystem
  Gain : Gain  Gain=0.007
  MPCControllerBlock : Subsystem  Commented=on  TreatAsAtomicUnit=on  SystemSampleTime=1
  MPCcontrollerEnable : Constant
  Memory1 : Memory  InitialCondition=refrigerant_p_init
  Memory{3,5..11} (8 alike) : Memory  InitialCondition=battery_T_init
  Memory2 : Memory  InitialCondition=refrigerant_p_init
  Memory4 : Memory  InitialCondition=1
  Preview : Subsystem
  Rate Transition{,1..2,4,7..10} (8 alike) : RateTransition  InitialCondition=battery_T_init  OutPortSampleTime=1
  Rate Transition3 : RateTransition  InitialCondition=1  OutPortSampleTime=1
  Rate Transition5 : RateTransition  InitialCondition=refrigerant_p_init  OutPortSampleTime=1
  Rate Transition6 : RateTransition  InitialCondition=refrigerant_p_init  OutPortSampleTime=1
  Scope{,1..16,19..40} (39 alike) : Scope
  Switch{1..8} (8 alike) : Switch  Criteria=u2 > Threshold  SaturateOnIntegerOverflow=off  InputSameDT=off
  T_battery : Subsystem
      mask Display: disp(get_param(gcb, 'Name'))
  Terminator : Terminator
  Thermal Mode : Subsystem
  Valves Control : Subsystem
  Zero-Order Hold{,1..5} (6 alike) : ZeroOrderHold  SampleTime=-1
  tag scope: CompressorSpd=global, MPCController=global, T_cabin_sp=global, T_vent_sp=global, batPumpNrpm=global, cabAirMfIn=global, cmd_battery_pump=global, cmd_blend_air=global, cmd_blower=global, cmd_comp=global, cmd_exv_chiller=global, cmd_exv_evap=global, cmd_exv_heatpump=global, cmd_fan=global, cmd_heater=global, cmd_motor_pump=global, cmd_parallel_serial=global, cmd_rad_bypass=global, cmd_recirc=global, cmd_refrig_bypass=global, heaterPwr=global, motPumpNrpm=global, radFanrpm=global, thermal_mode=global
  wires:
  [p_cond_evap_out] -> Fan Control/2(p_cond)
  [T_env] -> Fan Control/3(T_env)
  [T_inverter] -> Fan Control/5(T_inverter)
  [T_motor] -> Fan Control/6(T_motor)
  [T_env] -> Coolant Loop Control/2(T_env)
  Fan Control/1(cmd_fan) -> Scope26/1, [cmd_fan]
  Coolant Loop Control/2(cmd_motor_pump) -> Scope32/1, [cmd_motor_pump]
  Coolant Loop Control/3(cmd_battery_pump) -> Scope33/1, [cmd_battery_pump]
  [thermal_mode] -> Compressor Control/1(thermal_mode)
  Compressor Control/1(cmd_comp) -> Scope40/1, [cmd_comp]
  Cabin Air Control/1(cmd_blower) -> Scope27/1, [cmd_blower]
  Cabin Air Control/3(T_vent_sp) -> Scope30/1, [T_vent_sp]
  Valves Control/1(cmd_refrig_bypass) -> Scope34/1, [rule_cmdRefBypass]
  [T_motor] -> Coolant Loop Control/4(T_motor)
  [T_coolant_inverter_out] -> Coolant Loop Control/3(T_coolant_inverter_out)
  [cmd_comp] -> Fan Control/4(cmd_comp)
  [T_cabin] -> Cabin Air Control/1(T_cabin)
  [T_desired] -> Cabin Air Control/2(T_desired)
  [T_env] -> Cabin Air Control/3(T_env)
  Cabin Air Control/4(cmd_recirc) -> Scope29/1, [cmd_recirc]
  [v_vehicle] -> Fan Control/1(v_vehicle)
  [T_vent] -> Compressor Control/2(T_vent)
  [T_vent_sp] -> Compressor Control/3(T_vent_sp)
  [p_evap_out] -> Compressor Control/4(p_low)
  [p_inner_cond_out] -> Compressor Control/5(p_high)
  [thermal_mode] -> Coolant Loop Control/1(thermal_mode)
  Valves Control/2(cmd_blend_air) -> [rule_cmdBlendAir], Scope35/1
  Valves Control/6(cmd_exv_heatpump) -> Scope39/1, Scope15/1, Switch7/3
  Battery Heater Control/1(cmd_heater) -> Scope25/1, [cmd_heater]
  [T_coolant_battery_in] -> Battery Heater Control/2(T_coolant_battery_in)
  [T_env] -> Battery Heater Control/1(T_env)
  [T_env] -> Thermal Mode/1(T_env)
  [rpm_comp] -> Thermal Mode/2(rpm_comp)
  [T_coolant_inverter_out] -> Valves Control/2(T_coolant_inverter_out)
  [T_coolant_battery_in] -> Valves Control/3(T_coolant_battery_in)
  [T_env] -> Valves Control/4(T_env)
  [thermal_mode] -> Valves Control/1(thermal_mode)
  Thermal Mode/1(thermal_mode) -> Scope24/1, [internalThermal_mode]
  Cabin Air Control/2(T_cabin_sp) -> Scope28/1, [T_cabin_sp]
  [T_cabin] -> Rate Transition8/1
  T_battery/1(T_battery) -> [Tbat], Coolant Loop Control/5(T_battery)
  [T_cabInt] -> Rate Transition7/1
  Clock/1 -> Preview/2(Clock)
  [T_env] -> Preview/1(T_env)
  Preview/1(Tenv) -> Bus Creator/2
  Preview/2(MotHeat) -> Bus Creator/3
  Preview/3(InvHeat) -> Bus Creator/4
  Preview/4(DCDCHeat) -> Bus Creator/5
  Preview/5(BatteryCurrent) -> Bus Creator/6
  Preview/6(speed) -> Bus Creator/1
  Bus Creator/1 -> MPCControllerBlock/11(Preview)
  [T_coolant_inverter_out] -> Rate Transition9/1
  [T_coolant_battery_in] -> Rate Transition10/1
  [T_motor] -> Rate Transition/1
  [T_inverter] -> Rate Transition1/1
  [T_dcdc] -> Rate Transition2/1
  [SOC] -> Rate Transition3/1
  [Tbat] -> Rate Transition4/1
  MPCControllerBlock/1(Out1) -> Zero-Order Hold/1  "CompressorSpd"
  MPCControllerBlock/2(Out2) -> Zero-Order Hold1/1  "cabAirMfIn"
  MPCControllerBlock/3(Out3) -> Zero-Order Hold2/1
  MPCControllerBlock/4(Out4) -> Zero-Order Hold3/1
  [compPrIn] -> Rate Transition5/1
  Rate Transition/1 -> Memory7/1
  Rate Transition1/1 -> Memory6/1
  Rate Transition2/1 -> Memory5/1
  Rate Transition3/1 -> Memory4/1
  Rate Transition4/1 -> Memory3/1
  Rate Transition5/1 -> Memory1/1
  Rate Transition6/1 -> Memory2/1
  Rate Transition7/1 -> Memory8/1
  Rate Transition8/1 -> Memory9/1
  Rate Transition9/1 -> Memory10/1
  Rate Transition10/1 -> Memory11/1
  Memory1/1 -> MPCControllerBlock/6(compPrIn)
  Memory3/1 -> MPCControllerBlock/5(T_battery)
  Memory4/1 -> MPCControllerBlock/4(SOC)
  Memory6/1 -> MPCControllerBlock/2(T_inverter)
  Memory7/1 -> MPCControllerBlock/1(T_motor)
  Memory5/1 -> MPCControllerBlock/3(T_dcdc)
  Memory8/1 -> MPCControllerBlock/8(T_cabInt)
  Memory9/1 -> MPCControllerBlock/9(T_cabin)
  Memory10/1 -> MPCControllerBlock/12(T_coolant_inverter_out)
  Memory11/1 -> MPCControllerBlock/13(T_coolant_battery_in)
  MPCControllerBlock/5(Out5) -> Zero-Order Hold4/1
  Switch1/1 -> [thermal_mode]
  Switch2/1 -> [cmd_exv_chiller]
  Switch3/1 -> [cmd_parallel_serial]
  Switch4/1 -> [cmd_exv_evap]
  Switch5/1 -> [cmd_rad_bypass]
  Switch6/1 -> [cmd_blend_air]
  Switch7/1 -> [cmd_exv_heatpump]
  [internalThermal_mode] -> Scope1/1, Switch1/3
  [MPC_thermalMode] -> Scope/1, Switch1/1
  Switch8/1 -> [cmd_refrig_bypass]
  [MPC_cmdRefBypass] -> Scope4/1, Switch8/1
  [rule_cmdRefBypass] -> Scope5/1, Switch8/3
  [rule_cmdBlendAir] -> Scope6/1, Switch6/3
  [MPC_cmdBlendAir] -> Scope7/1, Switch6/1
  ControllerSwitch/1 -> Switch7/2, Switch3/2, Switch2/2, Switch6/2, Switch4/2, Switch8/2, Switch5/2, Switch1/2, [MPCController]
  [MPC_cmd_exv_chiller] -> Scope9/1, Switch2/1
  Valves Control/4(cmd_exv_chiller) -> [rule_cmd_exv_chiller], Scope37/1
  [rule_cmd_exv_chiller] -> Scope8/1, Switch2/3
  Valves Control/3(cmd_rad_bypass) -> [rule_cmd_rad_bypass], Scope36/1
  [rule_cmd_rad_bypass] -> Scope3/1, Switch5/3
  [MPC_cmdRadBypass] -> Scope2/1, Switch5/1
  Valves Control/5(cmd_exv_evap) -> Scope38/1, [rule_exvEvap]
  [rule_exvEvap] -> Scope11/1, Switch4/3
  [MPC_cmdExvEvap] -> Scope10/1, Switch4/1
  MPCControllerBlock/15(Out15) -> Gain/1
  Coolant Loop Control/1(cmd_parallel_serial) -> Scope31/1, Scope13/1, Switch3/3
  MPCControllerBlock/6(Out6) -> Zero-Order Hold5/1
  Gain/1 -> Scope14/1, Switch7/1
  MPCControllerBlock/9(Out9) -> [MPC_thermalMode]
  MPCControllerBlock/10(Out10) -> [MPC_cmdRefBypass]
  MPCControllerBlock/12(Out12) -> [MPC_cmdRadBypass]
  MPCControllerBlock/11(Out11) -> [MPC_cmdBlendAir]
  MPCControllerBlock/13(Out13) -> [MPC_cmd_exv_chiller]
  MPCControllerBlock/14(Out14) -> [MPC_cmdExvEvap]
  Memory2/1 -> MPCControllerBlock/7(compPrOut)
  [compPrOut] -> Rate Transition6/1
  Zero-Order Hold/1 -> Scope19/1, [CompressorSpd]
  Zero-Order Hold1/1 -> Scope20/1, [cabAirMfIn]
  Zero-Order Hold2/1 -> Scope21/1, [motPumpNrpm]
  Zero-Order Hold3/1 -> Scope22/1, [batPumpNrpm]
  Zero-Order Hold4/1 -> Scope23/1, [heaterPwr]
  Zero-Order Hold5/1 -> Scope16/1, [radFanrpm]
  [T_desired] -> Add/1
  Add/1 -> MPCControllerBlock/10(T_Cabdesired)
  Constant/1 -> Add/2
  [MPCController] -> MPCControllerBlock/14(MPCSwitch)
  Preview/7(mfCondEvap) -> Terminator/1

== system ElectricVehicleThermalManagementWithHeatPump/DCDC ==
  Controlled Heat Flow Rate Source : fl_lib/Thermal/Thermal Sources/Controlled Heat Flow Rate Source
  Coolant Jacket : SimscapeFluids_lib/Thermal Liquid/Pipes & Fittings/Pipe (TL)  dynamic_compressibility=simscape.enum.onoff.on  inertia=simscape.enum.onoff.off  num_segments=1  pipe_length=0.2 m  cross_section_geometry=fluids.thermal_liquid.pipes_fittings.enum.CrossSectionGeometry.Custom  pipe_diameter=0.1 m  pipe_inner_diameter=0.05 m  pipe_outer_diameter=0.1 m  pipe_width=0.1 m  pipe_height=0.1 m  pipe_major_axis=0.1 m  pipe_minor_axis=0.05 m  pipe_side=0.1 m  pipe_angle=30 deg  area=pi * coolant_channel_D^2 / 4 m^2  Dh=coolant_channel_D m  elevation_spec=foundation.enum.constant_variable.constant  elevation_gain=0 m  gravity_spec=foundation.enum.constant_variable.constant  g=9.81 m/s^2  pressure_loss_spec=fluids.thermal_liquid.pipes_fittings.enum.PressureLossSpec.Haaland  local_pressure_loss_spec=fluids.thermal_liquid.pipes_fittings.enum.LocalLossSpec.AggregateLength  length_add=0 m  loss_coefficient=0.1  roughness_spec=fluids.thermal_liquid.pipes_fittings.enum.RoughnessSpec.Custom  roughness=1.5e-5 m  Re_friction_TLU=[ 400 1000 1.5e+3 3e+3 4e+3 6e+3 1e+4 2e+4 4e+4 6e+4 1e+5 1e+8 ]  friction_factor_TLU=[ 0.264 0.112 0.07099999999999999 0.0417 0.0387 0.0268 0.025 0.0232 0.0226 0.022 0.0214 0.0214 ]  Re_lam=100  Re_tur=500  shape_factor=64  mdot_nominal=[ 0.1 1 ] kg/s  p_diff_nominal=[ 0.001 0.01 ] MPa  mdot_threshold=1e-6 kg/s  wall_spec=fluids.thermal_liquid.pipes_fittings.enum.wall_spec.rigid  vol_expansion_spec=fluids.thermal_liquid.pipes_fittings.enum.VolumeExpansionSpec.Diameter  area_pressure_gain=1e-6 m^2/MPa  static_pressure_TLU=[.1, 1] MPa  area_pressure_gain_TLU=[1e-05, 1.1e-05] m^2  material_behavior_spec=fluids.thermal_liquid.pipes_fittings.enum.PipeMaterialBehavior.Linear  diameter_pressure_gain=1.2e-6 m/MPa  wall_thickness=0.05 m  elastic_modulus=69 GPa  stress_TLU=[276, 310] MPa  strain_TLU=[.004, .02]  stress_assert_action=simscape.enum.assert.action.none  stress_max=400 MPa  poisson_ratio=0.33  wall_time_constant=0.01 s  thermal_expansion=false  alpha_L_wall=24 um/(deltaK*m)  thermal_expansion_Tref=293.15 K  heat_transfer_spec=fluids.thermal_liquid.pipes_fittings.enum.HeatTransferSpec.DittusBoelter  mdot_nominal_heat=[ 0.1 1 ] kg/s  T_in_nominal=[ 293.15 293.15 ] K  T_out_nominal=[ 300 300 ] K  p_in_nominal_heat=[ 0.101325 0.101325 ] MPa  T_wall_nominal=[ 303.15 303.15 ] K  a_coeff=0.3  b_Re_power=0.8  c_Pr_power=0.33  Nu_lam=3.66  Re_Colburn_TLU=[ 100 150 1000 ]  Colburn_factor_TLU=[ 0.019 0.013 0.002 ]  Re_Nu_TLU=[ 100 150 1000 ]  Pr_Nu_TLU=[ 1 10 ]  Nu_TLU=[ 3.72 4.21; 3.75 4.44; 4.21 7.15 ]  p0_vec=coolant_p_init MPa  T0_vec=coolant_T_init degC  mdot0=0.1 kg/s
  DC-DC Converter : fl_lib/Thermal/Thermal Elements/Thermal Mass  mass_type=foundation.enum.constant_variable.constant  mass=1 kg  sp_heat=447 J/kg/K  mass_min=1e-6 kg  num_ports=foundation.enum.numPorts2.one  m_specify=off  m_priority=High  m=1 kg  m_nominal_specify=off  m_nominal_value=1  m_nominal_unit=kg  T_specify=on  T_priority=High  T=coolant_T_init degC  T_nominal_specify=off  T_nominal_value=1  T_nominal_unit=K  Q_specify=off  Q_priority=None  Q=0 W  Q_nominal_specify=off  Q_nominal_value=1  Q_nominal_unit=W
  Flow Rate Sensor (TL) : fl_lib/Thermal Liquid/Sensors/Flow Rate Sensor (TL)  mass_flow_measure=true  volumetric_flow_measure=false  energy_flow_measure=true
      settings: InternalSimscapePortConfiguration="{\"Bottom\":[{\"id\":\"PHI\",\"label\":\"φ\",\"type\":\"output\"}],\"Left\":[{\"id\":\"A\",\"label\":\"A\",\"type\":\"foundation.thermal_liquid.thermal_liquid\"}],\"Right\":[{\"id\":\"B\",\"label\":\"B\",\"type\":\"foundation.thermal_liquid.thermal_liquid\"},{\"id\":\"M\",\"label\":\"M\",\"type\":\"output\"}],\"Top\":[]}"
  Flow Resistance (TL) : fl_lib/Thermal Liquid/Elements/Flow Resistance (TL)  delta_p_nominal=2e-3 MPa  mdot_nominal=0.02 kg/s  area=pi * coolant_pipe_D^2 / 4 m^2  laminar_fraction=1e-3
  Flow Resistance (TL)1 : fl_lib/Thermal Liquid/Elements/Flow Resistance (TL)  delta_p_nominal=1e-5 MPa  mdot_nominal=0.02 kg/s  area=pi * coolant_pipe_D^2 / 4 m^2  laminar_fraction=1e-3
  PS-Simulink Converter : nesl_utility/PS-Simulink Converter  PhysicalDomain=network_engine_domain  SubClassName=ps_output  LeftPortType=input  RightPortType=output  PseudoPeriodic=off  Frequencies=[]  VectorFormat=inherit  Unit=degC  AffineConversion=on
  PS-Simulink Converter1 : nesl_utility/PS-Simulink Converter  PhysicalDomain=network_engine_domain  SubClassName=ps_output  LeftPortType=input  RightPortType=output  PseudoPeriodic=off  Frequencies=[]  VectorFormat=inherit  Unit=inherit  AffineConversion=off
  Scope : Scope
  Simulink-PS Converter : nesl_utility/Simulink-PS Converter  PhysicalDomain=network_engine_domain  SubClassName=ps_input  LeftPortType=input  RightPortType=output  PseudoPeriodic=off  Frequencies=[]  NoiseDistribution=none  NoiseParameters=[]  Unit=W  AffineConversion=off  FilteringAndDerivatives=provide  SimscapeFilterOrder=1  InputFilterTimeConstant=0.001  UdotUserProvided=0
  Temperature Sensor : fl_lib/Thermal/Thermal Sensors/Temperature Sensor  temperature_measure=foundation.enum.MeasurementReference.absolute
      settings: InternalSimscapePortConfiguration="{\"Bottom\":[],\"Left\":[{\"id\":\"A\",\"label\":\"A\",\"type\":\"foundation.thermal.thermal\"}],\"Right\":[{\"id\":\"T\",\"label\":\"T\",\"type\":\"output\"}],\"Top\":[]}"
  Thermal Reference : fl_lib/Thermal/Thermal Elements/Thermal Reference
  To Workspace : ToWorkspace  VariableName=mf_dcdc  SampleTime=-1
  To Workspace1 : ToWorkspace  VariableName=Q_dcdcMeasured  SampleTime=-1
  To Workspace2 : ToWorkspace  VariableName=T_dcdcMeas  SampleTime=-1
  B : PMIOPort  Side=Left
  A : PMIOPort  Port=2  Side=Right
  tag scope: T_dcdc=global
  wires:
  [Q_dcdc] -> To Workspace1/1, Simulink-PS Converter/1
  PS-Simulink Converter/1 -> To Workspace2/1, [T_dcdc]
  PS-Simulink Converter1/1 -> To Workspace/1, Scope/1
  connections:
  Coolant Jacket/LConn2 -- Controlled Heat Flow Rate Source/LConn1 -- Temperature Sensor/LConn1 -- DC-DC Converter/LConn1
  PS-Simulink Converter/LConn1 -- Temperature Sensor/RConn1
  Controlled Heat Flow Rate Source/RConn2 -- Thermal Reference/LConn1
  Simulink-PS Converter/RConn1 -- Controlled Heat Flow Rate Source/RConn1
  Coolant Jacket/LConn1 -- Flow Rate Sensor (TL)/RConn1
  PS-Simulink Converter1/LConn1 -- Flow Rate Sensor (TL)/RConn2
  Flow Resistance (TL)/LConn1 -- A/RConn1
  Flow Resistance (TL)/RConn1 -- Flow Rate Sensor (TL)/LConn1
  Flow Resistance (TL)1/LConn1 -- Coolant Jacket/RConn1
  Flow Resistance (TL)1/RConn1 -- B/RConn1
